simulink model "AvonGasTurbineController"  (R2024b)
settings: Solver=ode45  StartTime=0.0  StopTime=3000  FixedStep=1  RelTol=1e-3  EnableMultiTasking=on
InitFcn:
  | warning off
libraries: slpidlib x3, simulink x2
(part 1 of 2)
settings Model: Creator=Me  LastModifiedBy=argha
settings SolverCC: AlgebraicLoopSolver=TrustRegion
settings DataIOCC: LimitDataPoints=on  SaveFormat=Array  SignalLoggingSaveFormat=ModelDataLogs  ReturnWorkspaceOutputs=off
settings OptimizationCC: ExpressionDepthLimit=2147483647  LifeSpan=inf
settings DebuggingCC: UnderspecifiedInitializationDetection=Classic  MergeDetectMultiDrivingBlocksExec=none  SolverPrmCheckMsg=warning  FcnCallInpInsideContextMsg=warning  UnconnectedInputMsg=warning  UnconnectedOutputMsg=warning  UnconnectedLineMsg=warning  StateNameClashWarn=warning  SFUnexpectedBacktrackingDiag=warning  SFNoUnconditionalDefaultTransitionDiag=warning  SFExecutionAtInitializationDiag=none  ArithmeticOperatorsInVariantConditions=warning
settings HardwareCC: ProdBitPerPointer=32  ProdBitPerSizeT=32  ProdBitPerPtrDiffT=32  ProdLargestAtomicFloat=None  ProdIntDivRoundTo=Undefined  ProdEndianess=Unspecified  ProdWordSize=32  ProdHWDeviceType=32-bit Generic
settings ModelReferenceCC: EnableRefExpFcnMdlSchedulingChecks=on  PropagateSignalLabelsOutOfModel=off
settings SFSimCC: SimUseLocalCustomCode=off  CustomCodeUndefinedFunction=UseInterfaceOnly
settings RTWCC: RTWUseLocalCustomCode=off  GPUComputeCapability=3.5
settings CodeAppCC: StateflowObjectComments=on
settings GRTTargetCC: TargetLangStandard=C89/C90 (ANSI)  CombineOutputUpdateFcns=off  GRTInterface=on
settings ConfigComp: CovMetricSettings=dw  CovSaveCumulativeToWorkspaceVar=on  CovSaveSingleToWorkspaceVar=on  CovExternalEMLEnable=off  CovSFcnEnable=off
settings SimscapeCC: SimscapeNormalizeSystem=off
settings ConfigurationSet: Description=SimMechanics 2G

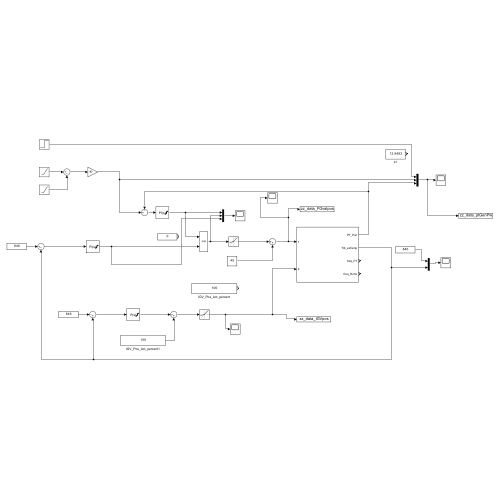
[thumbnail: Simulink's stored preview of the top-level diagram]
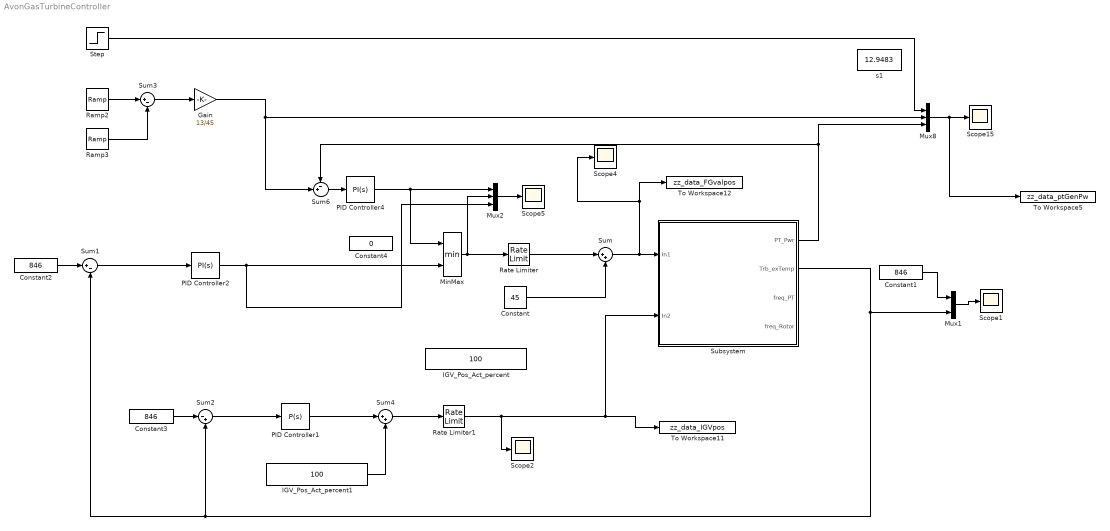
== system AvonGasTurbineController ==
  Constant : Constant  Value=45
  Constant1 : Constant  Value=846
  Constant2 : Constant  Value=846
  Constant3 : Constant  Value=846
  Constant4 : Constant  Value=0
  Gain : Gain  Gain=13/45
  IGV_Pos_Act_percent : Constant  Value=100
  IGV_Pos_Act_percent1 : Constant  Value=100
  MinMax : MinMax  Inputs=2
  Mux1 : Mux  Inputs=2
  Mux2 : Mux  Inputs=3
  Mux8 : Mux  Inputs=3
  PID Controller1 : slpidlib/PID Controller  Controller=P  Form=Ideal  TimeDomain=Continuous-time  UseExternalTs=off  SampleTime=-1  IntegratorMethod=Forward Euler  FilterMethod=Forward Euler  ControllerParametersSource=internal  P=0.1  I=0.180070827922895  UseKiTs=off  D=0  UseExternalDerivativeSource=off  N=100  UseFilter=on  TunerSelectOption=Transfer Function Based (PID Tuner App)  InitialConditionSource=internal  InitialConditionForIntegrator=0  InitialConditionForFilter=0  DifferentiatorICPrevScaledInput=0  ExternalReset=none  TrackingMode=off  Kt=1  LimitOutput=on  SatLimitsSource=internal  UpperSaturationLimit=15  LowerSaturationLimit=-100  LinearizeAsGain=on  AntiWindupMode=back-calculation  Kb=0.2  LimitIntegrator=off  UpperIntegratorSaturationLimit=inf  LowerIntegratorSaturationLimit=-inf  POutMin=[]  POutMax=[]  IOutMin=[]  IOutMax=[]  DOutMin=[]  DOutMax=[]  NOutMin=[]  NOutMax=[]  SumOutMin=[]  SumOutMax=[]  SaturationOutMin=[]  SaturationOutMax=[]  PParamMin=[]  PParamMax=[]  IParamMin=[]  IParamMax=[]  DParamMin=[]  DParamMax=[]  NParamMin=[]  NParamMax=[]  KbParamMin=[]  KbParamMax=[]  KtParamMin=[]  KtParamMax=[]  KbOutMin=[]  KbOutMax=[]  KtOutMin=[]  KtOutMax=[]  IntegratorOutMin=[]  IntegratorOutMax=[]  FilterOutMin=[]  FilterOutMax=[]  SumI1OutMin=[]  SumI1OutMax=[]  SumI2OutMin=[]  SumI2OutMax=[]  SumI3OutMin=[]  SumI3OutMax=[]  SumI4OutMin=[]  SumI4OutMax=[]  SumDOutMin=[]  SumDOutMax=[]  DifferentiatorOutMin=[]  DifferentiatorOutMax=[]  FilterDiffOutCoefMin=[]  FilterDiffOutCoefMax=[]  ReciprocalOutMin=[]  ReciprocalOutMax=[]  SumDenOutMin=[]  SumDenOutMax=[]  SumNumOutMin=[]  SumNumOutMax=[]  DivideOutMin=[]  DivideOutMax=[]  UdiffTsProdOutMin=[]  UdiffTsProdOutMax=[]  NTsProdOutMin=[]  NTsProdOutMax=[]  UintegralTsProdOutMin=[]  UintegralTsProdOutMax=[]  UngainTsProdOutMin=[]  UngainTsProdOutMax=[]  ClampingZeroOutDataTypeStr=Inherit: Inherit via back propagation  ClampingZeroOutMin=[]  ClampingZeroOutMax=[]  FilterDenConstantOutDataTypeStr=Inherit: Inherit via back propagation  FilterDenConstantOutMin=[]  FilterDenConstantOutMax=[]  PCopyOutDataTypeStr=Inherit: Inherit via back propagation  PCopyOutMin=[]  PCopyOutMax=[]  NCopyOutDataTypeStr=Inherit: Inherit via back propagation  NCopyOutMin=[]  NCopyOutMax=[]  IntegratorContinuousStateAttributes=''  IntegratorStateMustResolveToSignalObject=off  IntegratorRTWStateStorageClass=Auto  FilterContinuousStateAttributes=''  FilterStateMustResolveToSignalObject=off  FilterRTWStateStorageClass=Auto  ParallelPVariant=InternalParameters  IdealPVariant=Disabled  IVariant=Disabled  DVariant=Disabled  IntegratorVariant=Disabled  SatVariant=Enabled  AWVariant=Disabled  PCopyVariant=Disabled  TRVariant=Disabled  FdbkBlocksVariant=Forward  IdealPFdbkVariant=Disabled  SatFdbkVariant=Disabled  DerivativeFilterVariant=Disabled  NVariant=Disabled  NCopyVariant=Disabled_SignalSpec  FilterICVariant=Disabled  IntegratorICVariant=Disabled  ExternalResetVariant=Disabled  TRSumVariant=Passthrough  SumFdbkVariant=Disabled  SumVariant=Passthrough_P  TsampFilterVariant=InternalTs  TsampNgainVariant=Passthrough  TsampIntegralVariant=Disabled_SignalSpec  ExternalSaturationOutDataTypeStr=Inherit: Same as second input  DerivativeSourceVariant=Disabled  PreIntVariant=InternalPreInt
  PID Controller2 : slpidlib/PID Controller  Controller=PI  Form=Ideal  TimeDomain=Continuous-time  UseExternalTs=off  SampleTime=-1  IntegratorMethod=Forward Euler  FilterMethod=Forward Euler  ControllerParametersSource=internal  P=0.02  I=0.1  UseKiTs=off  D=0  UseExternalDerivativeSource=off  N=100  UseFilter=on  TunerSelectOption=Transfer Function Based (PID Tuner App)  InitialConditionSource=internal  InitialConditionForIntegrator=20  InitialConditionForFilter=0  DifferentiatorICPrevScaledInput=0  ExternalReset=none  TrackingMode=off  Kt=1  LimitOutput=on  SatLimitsSource=internal  UpperSaturationLimit=45  LowerSaturationLimit=-45  LinearizeAsGain=on  AntiWindupMode=back-calculation  Kb=0.2  LimitIntegrator=off  UpperIntegratorSaturationLimit=inf  LowerIntegratorSaturationLimit=-inf  POutMin=[]  POutMax=[]  IOutMin=[]  IOutMax=[]  DOutMin=[]  DOutMax=[]  NOutMin=[]  NOutMax=[]  SumOutMin=[]  SumOutMax=[]  SaturationOutMin=[]  SaturationOutMax=[]  PParamMin=[]  PParamMax=[]  IParamMin=[]  IParamMax=[]  DParamMin=[]  DParamMax=[]  NParamMin=[]  NParamMax=[]  KbParamMin=[]  KbParamMax=[]  KtParamMin=[]  KtParamMax=[]  KbOutMin=[]  KbOutMax=[]  KtOutMin=[]  KtOutMax=[]  IntegratorOutMin=[]  IntegratorOutMax=[]  FilterOutMin=[]  FilterOutMax=[]  SumI1OutMin=[]  SumI1OutMax=[]  SumI2OutMin=[]  SumI2OutMax=[]  SumI3OutMin=[]  SumI3OutMax=[]  SumI4OutMin=[]  SumI4OutMax=[]  SumDOutMin=[]  SumDOutMax=[]  DifferentiatorOutMin=[]  DifferentiatorOutMax=[]  FilterDiffOutCoefMin=[]  FilterDiffOutCoefMax=[]  ReciprocalOutMin=[]  ReciprocalOutMax=[]  SumDenOutMin=[]  SumDenOutMax=[]  SumNumOutMin=[]  SumNumOutMax=[]  DivideOutMin=[]  DivideOutMax=[]  UdiffTsProdOutMin=[]  UdiffTsProdOutMax=[]  NTsProdOutMin=[]  NTsProdOutMax=[]  UintegralTsProdOutMin=[]  UintegralTsProdOutMax=[]  UngainTsProdOutMin=[]  UngainTsProdOutMax=[]  ClampingZeroOutDataTypeStr=Inherit: Inherit via back propagation  ClampingZeroOutMin=[]  ClampingZeroOutMax=[]  FilterDenConstantOutDataTypeStr=Inherit: Inherit via back propagation  FilterDenConstantOutMin=[]  FilterDenConstantOutMax=[]  PCopyOutDataTypeStr=Inherit: Inherit via back propagation  PCopyOutMin=[]  PCopyOutMax=[]  NCopyOutDataTypeStr=Inherit: Inherit via back propagation  NCopyOutMin=[]  NCopyOutMax=[]  IntegratorContinuousStateAttributes=''  IntegratorStateMustResolveToSignalObject=off  IntegratorRTWStateStorageClass=Auto  FilterContinuousStateAttributes=''  FilterStateMustResolveToSignalObject=off  FilterRTWStateStorageClass=Auto  ParallelPVariant=Passthrough  IdealPVariant=InternalParameters  IVariant=InternalParameters  DVariant=Disabled  IntegratorVariant=Continuous  SatVariant=Enabled  AWVariant=BackCalculation  PCopyVariant=Disabled  TRVariant=Disabled  FdbkBlocksVariant=Forward  IdealPFdbkVariant=Disabled  SatFdbkVariant=Disabled  DerivativeFilterVariant=Disabled  NVariant=Disabled  NCopyVariant=Disabled_SignalSpec  FilterICVariant=Disabled  IntegratorICVariant=InternalICs  ExternalResetVariant=Disabled  TRSumVariant=Passthrough  SumFdbkVariant=Disabled  SumVariant=Sum_PI  TsampFilterVariant=InternalTs  TsampNgainVariant=Passthrough  TsampIntegralVariant=Disabled_SignalSpec  ExternalSaturationOutDataTypeStr=Inherit: Same as second input  DerivativeSourceVariant=Disabled  PreIntVariant=InternalPreInt
  PID Controller4 : slpidlib/PID Controller  Controller=PI  Form=Ideal  TimeDomain=Continuous-time  UseExternalTs=off  SampleTime=-1  IntegratorMethod=Forward Euler  FilterMethod=Forward Euler  ControllerParametersSource=internal  P=0.17  I=0.2  UseKiTs=off  D=0  UseExternalDerivativeSource=off  N=100  UseFilter=on  TunerSelectOption=Transfer Function Based (PID Tuner App)  InitialConditionSource=internal  InitialConditionForIntegrator=0  InitialConditionForFilter=0  DifferentiatorICPrevScaledInput=0  ExternalReset=none  TrackingMode=off  Kt=1  LimitOutput=on  SatLimitsSource=internal  UpperSaturationLimit=60  LowerSaturationLimit=-30  LinearizeAsGain=on  AntiWindupMode=back-calculation  Kb=0.2  LimitIntegrator=off  UpperIntegratorSaturationLimit=inf  LowerIntegratorSaturationLimit=-inf  POutMin=[]  POutMax=[]  IOutMin=[]  IOutMax=[]  DOutMin=[]  DOutMax=[]  NOutMin=[]  NOutMax=[]  SumOutMin=[]  SumOutMax=[]  SaturationOutMin=[]  SaturationOutMax=[]  PParamMin=[]  PParamMax=[]  IParamMin=[]  IParamMax=[]  DParamMin=[]  DParamMax=[]  NParamMin=[]  NParamMax=[]  KbParamMin=[]  KbParamMax=[]  KtParamMin=[]  KtParamMax=[]  KbOutMin=[]  KbOutMax=[]  KtOutMin=[]  KtOutMax=[]  IntegratorOutMin=[]  IntegratorOutMax=[]  FilterOutMin=[]  FilterOutMax=[]  SumI1OutMin=[]  SumI1OutMax=[]  SumI2OutMin=[]  SumI2OutMax=[]  SumI3OutMin=[]  SumI3OutMax=[]  SumI4OutMin=[]  SumI4OutMax=[]  SumDOutMin=[]  SumDOutMax=[]  DifferentiatorOutMin=[]  DifferentiatorOutMax=[]  FilterDiffOutCoefMin=[]  FilterDiffOutCoefMax=[]  ReciprocalOutMin=[]  ReciprocalOutMax=[]  SumDenOutMin=[]  SumDenOutMax=[]  SumNumOutMin=[]  SumNumOutMax=[]  DivideOutMin=[]  DivideOutMax=[]  UdiffTsProdOutMin=[]  UdiffTsProdOutMax=[]  NTsProdOutMin=[]  NTsProdOutMax=[]  UintegralTsProdOutMin=[]  UintegralTsProdOutMax=[]  UngainTsProdOutMin=[]  UngainTsProdOutMax=[]  ClampingZeroOutDataTypeStr=Inherit: Inherit via back propagation  ClampingZeroOutMin=[]  ClampingZeroOutMax=[]  FilterDenConstantOutDataTypeStr=Inherit: Inherit via back propagation  FilterDenConstantOutMin=[]  FilterDenConstantOutMax=[]  PCopyOutDataTypeStr=Inherit: Inherit via back propagation  PCopyOutMin=[]  PCopyOutMax=[]  NCopyOutDataTypeStr=Inherit: Inherit via back propagation  NCopyOutMin=[]  NCopyOutMax=[]  IntegratorContinuousStateAttributes=''  IntegratorStateMustResolveToSignalObject=off  IntegratorRTWStateStorageClass=Auto  FilterContinuousStateAttributes=''  FilterStateMustResolveToSignalObject=off  FilterRTWStateStorageClass=Auto  ParallelPVariant=Passthrough  IdealPVariant=InternalParameters  IVariant=InternalParameters  DVariant=Disabled  IntegratorVariant=Continuous  SatVariant=Enabled  AWVariant=BackCalculation  PCopyVariant=Disabled  TRVariant=Disabled  FdbkBlocksVariant=Forward  IdealPFdbkVariant=Disabled  SatFdbkVariant=Disabled  DerivativeFilterVariant=Disabled  NVariant=Disabled  NCopyVariant=Disabled_SignalSpec  FilterICVariant=Disabled  IntegratorICVariant=InternalICs  ExternalResetVariant=Disabled  TRSumVariant=Passthrough  SumFdbkVariant=Disabled  SumVariant=Sum_PI  TsampFilterVariant=InternalTs  TsampNgainVariant=Passthrough  TsampIntegralVariant=Disabled_SignalSpec  ExternalSaturationOutDataTypeStr=Inherit: Same as second input  DerivativeSourceVariant=Disabled  PreIntVariant=InternalPreInt
  Ramp2 : simulink/Sources/Ramp  slope=0.05  start=1500  InitialOutput=30
  Ramp3 : simulink/Sources/Ramp  slope=0.05  start=1800  InitialOutput=0
  Rate Limiter : RateLimiter  RisingSlewLimit=0.1  FallingSlewLimit=-0.1  SampleTimeMode=inherited  InitialCondition=45
  Rate Limiter1 : RateLimiter  RisingSlewLimit=0.1  FallingSlewLimit=-0.1  SampleTimeMode=inherited  InitialCondition=45
  Scope{1..2,4..5,15} (5 alike) : Scope
  Step : Step  Time=1500  Before=8.66  After=13  SampleTime=0
  Subsystem : Subsystem
  Sum : Sum  Inputs=|++
  Sum1 : Sum  Inputs=|+-
  Sum2 : Sum  Inputs=|-+
  Sum3 : Sum  Inputs=|+-
  Sum4 : Sum  Inputs=|++
  Sum6 : Sum  Inputs=-+|
  To Workspace11 : ToWorkspace  VariableName=zz_data_IGVpos  SampleTime=1
  To Workspace12 : ToWorkspace  VariableName=zz_data_FGvalpos  SampleTime=1
  To Workspace5 : ToWorkspace  VariableName=zz_data_ptGenPw  SampleTime=1
  s1 : Constant  Value=12.9483
  wires:
  Ramp3/1 -> Sum3/2
  Ramp2/1 -> Sum3/1
  Subsystem/2(Trb_exTemp) -> Mux1/2, Sum2/2, Sum1/2
  Sum3/1 -> Gain/1
  Sum6/1 -> PID Controller4/1
  Constant2/1 -> Sum1/1
  PID Controller2/1 -> Mux2/3, MinMax/2
  PID Controller4/1 -> Mux2/1, MinMax/1
  Gain/1 -> Mux8/2, Sum6/2
  Constant/1 -> Sum/2
  Sum/1 -> Scope4/1, To Workspace12/1, Subsystem/1(In1)
  MinMax/1 -> Mux2/2, Rate Limiter/1
  Mux1/1 -> Scope1/1
  Constant1/1 -> Mux1/1
  Sum2/1 -> PID Controller1/1
  Constant3/1 -> Sum2/1
  PID Controller1/1 -> Sum4/1
  IGV_Pos_Act_percent1/1 -> Sum4/2
  Sum4/1 -> Rate Limiter1/1
  Rate Limiter1/1 -> Subsystem/2(In2), To Workspace11/1, Scope2/1
  Mux8/1 -> To Workspace5/1, Scope15/1
  Subsystem/1(PT_Pwr) -> Mux8/3, Sum6/1
  Step/1 -> Mux8/1
  Sum1/1 -> PID Controller2/1
  Rate Limiter/1 -> Sum/1
  Mux2/1 -> Scope5/1

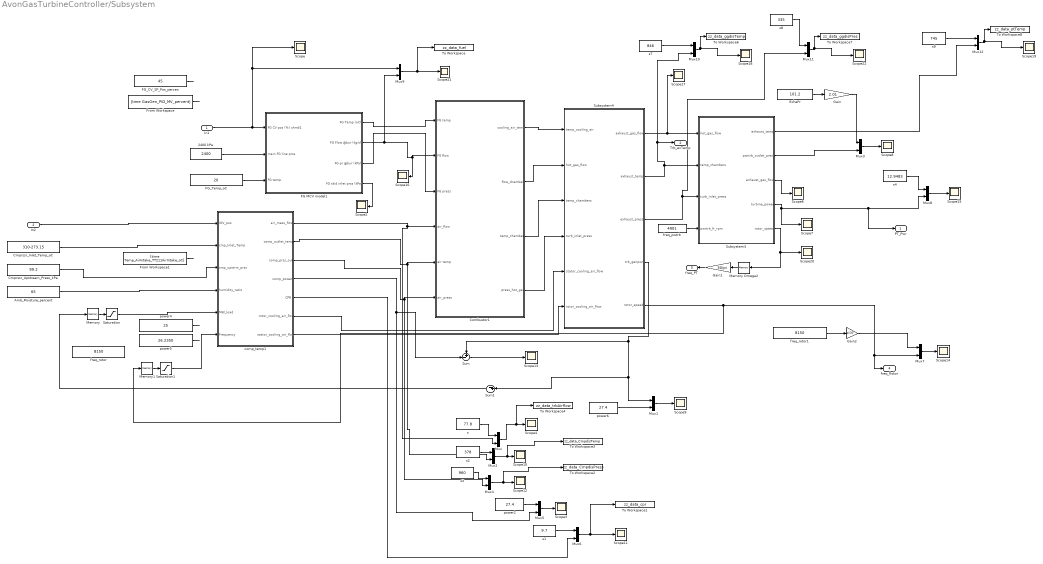
== system AvonGasTurbineController/Subsystem ==
  In1 : Inport
  In2 : Inport  Port=2
  2400 kPa : Constant  Value=2400
  Amb_Moisture_percent : Constant  Value=65
  Cmprssr_Inlet_Temp_oC : Constant  Value=310-273.15
  Cmprssr_Upstream_Press_kPa : Constant  Value=99.2
  Combustor1 : Subsystem
  ExhaPr : Constant  Value=101.2
  FG MCV model1 : Subsystem
  FG_CV_SP_Pos_percen : Constant  Value=45
  FG_Temp_oC : Constant  Value=20
  From Workspace : FromWorkspace  VariableName=[time GasGen_PID_MV_percent]
  From Workspace1 : FromWorkspace  VariableName="[time  Temp_AirIntake_TT211AirIntake_oC]"
  Gain : Gain  Gain=2.01
  Gain1 : Gain  Gain=30/pi
  Gain2 : Gain  Gain=pi/30
  Memory : Memory  InitialCondition=28.945
  Memory Omega2 : Memory  InitialCondition=pi/30*4901
  Memory1 : Memory  InitialCondition=8150
  Mux{,1..12} (13 alike) : Mux  Inputs=2
  Saturation : Saturate  UpperLimit=40  LowerLimit=1
  Saturation1 : Saturate  UpperLimit=8300  LowerLimit=7000
  Scope{,2..4,6..22} (21 alike) : Scope
  Subsystem3 : Subsystem
  Subsystem4 : Subsystem
  Sum : Sum  Inputs=+-|
  Sum1 : Sum  Inputs=-+|
  To Workspace : ToWorkspace  VariableName=zz_data_fuel  SaveFormat=Timeseries  SampleTime=1
  To Workspace1 : ToWorkspace  VariableName=zz_data_cpr  SampleTime=1
  To Workspace2 : ToWorkspace  VariableName=zz_data_CmpdisPress  SampleTime=1
  To Workspace3 : ToWorkspace  VariableName=zz_data_CmpdisTemp  SaveFormat=Timeseries  SampleTime=1
  To Workspace4 : ToWorkspace  VariableName=zz_data_trbAirflow  SampleTime=1
  To Workspace6 : ToWorkspace  VariableName=zz_data_ggdisTemp  SampleTime=1
  To Workspace7 : ToWorkspace  VariableName=zz_data_ggdisPres  SampleTime=1
  To Workspace8 : ToWorkspace  VariableName=zz_data_ptTemp  SampleTime=1
  comp_temp1 : Subsystem
  freq_pwtrb : Constant  Value=4901
  freq_rotor : Constant  Value=8150
  freq_rotor1 : Constant  Value=8150
  power2 : Constant  Value=27.4
  power4 : Constant  Value=25
  power5 : Constant  Value=26.2350
  power6 : Constant  Value=27.4
  s : Constant  Value=77.8
  s1 : Constant  Value=9.7
  s2 : Constant  Value=378
  s3 : Constant  Value=960
  s4 : Constant  Value=12.9483
  s7 : Constant  Value=846
  s8 : Constant  Value=335
  s9 : Constant  Value=745
  PT_Pwr : Outport
  Trb_exTemp : Outport  Port=2
  freq_PT : Outport  Port=3
  freq_Rotor : Outport  Port=4
  wires:
  FG_CV_SP_Pos_percen/1 -> ?
  From Workspace/1 -> ?
  Gain1/1 -> freq_PT/1
  From Workspace1/1 -> ?
  power5/1 -> ?
  power4/1 -> ?
  Subsystem4/2(exhaust_temp) -> Subsystem3/2(temp_chambers), Trb_exTemp/1, Mux10/2
  Cmprssr_Upstream_Press_kPa/1 -> comp_temp1/3(cmp_upstrm_prss)
  Amb_Moisture_percent/1 -> comp_temp1/4(humidity_ratio)
  Saturation1/1 -> comp_temp1/6(Frequency)
  In2/1 -> comp_temp1/1(IGV_pos)
  Subsystem3/3(exhaust_gas_flow) -> Scope6/1
  Memory/1 -> Saturation/1
  FG_Temp_oC/1 -> FG MCV model1/3(FG temp.)
  comp_temp1/3(comp_prss_out) -> Mux4/2, Combustor1/6(air_press)
  FG MCV model1/2(FG Flow @bur (kg/s)) -> Mux9/2, Scope16/1, Combustor1/2(FG flow)
  Combustor1/2(flow_chamber) -> Subsystem4/2(hot_gas_flow)
  comp_temp1/4(comp_power) -> Mux5/2, Sum/2
  Mux1/1 -> Scope9/1
  Mux6/1 -> To Workspace1/1, Scope11/1
  comp_temp1/5(CPR) -> Mux6/2
  Mux4/1 -> To Workspace2/1, Scope12/1
  FG MCV model1/1(FG Temp (oC)) -> Combustor1/1(FG temp)
  Mux2/1 -> To Workspace3/1, Scope10/1
  2400 kPa/1 -> FG MCV model1/2(main FG line prss)
  ExhaPr/1 -> Gain/1
  Combustor1/1(cooling_air_temp) -> Subsystem4/1(temp_cooling_air)
  FG MCV model1/3(FG pr @bur (kPa)) -> Combustor1/3(FG press)
  Subsystem4/3(exhaust_press) -> Mux11/2, Subsystem3/3(turb_inlet_press)
  Combustor1/3(temp_chamber) -> Subsystem4/3(temp_chambers)
  FG MCV model1/4(FG skid inlet prss (kPa)) -> Scope2/1
  Subsystem4/1(exhaust_gas_flow) -> Scope17/1, Subsystem3/1(hot_gas_flow)
  Subsystem3/2(pwrtrb_outlet_press) -> Mux3/2
  power6/1 -> Mux1/2
  Gain/1 -> Mux3/1
  Mux3/1 -> Scope8/1
  comp_temp1/1(air_mass_flow) -> Mux/2, Combustor1/4(air_flow)
  Subsystem3/1(exhaust_temp) -> Mux12/2
  comp_temp1/2(comp_outlet_temp) -> Mux2/2, Combustor1/5(air temp)
  Combustor1/4(press_hot_gas) -> Subsystem4/4(turb_inlet_press)
  Mux8/1 -> Scope15/1
  Mux7/1 -> Scope14/1
  In1/1 -> Mux9/1, Scope/1, FG MCV model1/1(FG CV pos (%) chmb1)
  Subsystem3/4(turbine_power) -> PT_Pwr/1, Mux8/2, Scope7/1
  comp_temp1/7(stator_cooling_air_flow) -> Subsystem4/6(rotor_cooling_air_flow)
  Cmprssr_Inlet_Temp_oC/1 -> comp_temp1/2(cmp_Inlet_Temp)
  Mux11/1 -> To Workspace7/1, Scope22/1
  s2/1 -> Mux2/1
  Sum1/1 -> Memory/1
  Mux9/1 -> To Workspace/1, Scope21/1
  Mux/1 -> To Workspace4/1, Scope4/1
  s/1 -> Mux/1
  s7/1 -> Mux10/1
  s1/1 -> Mux6/1
  Mux10/1 -> Scope18/1, To Workspace6/1
  Mux5/1 -> Scope3/1
  Sum/1 -> Scope13/1
  Subsystem4/5(rotor_speed) -> Memory1/1, freq_Rotor/1, Mux7/2
  comp_temp1/6(rotor_cooling_air_flow) -> Subsystem4/5(stator_cooling_air_flow)
  s3/1 -> Mux4/1
  freq_pwtrb/1 -> Subsystem3/4(pwrtrb_fr_rpm)
  power2/1 -> Mux5/1
  Subsystem3/5(rotor_speed) -> Scope20/1, Memory Omega2/1
  Gain2/1 -> Mux7/1
  Saturation/1 -> comp_temp1/5(MW_load)
  Memory Omega2/1 -> Gain1/1
  freq_rotor1/1 -> Gain2/1
  Subsystem4/4(trb_genpwr) -> Sum/1, Sum1/2, Mux1/1
  s4/1 -> Mux8/1
  s9/1 -> Mux12/1
  s8/1 -> Mux11/1
  Mux12/1 -> To Workspace8/1, Scope19/1
  Memory1/1 -> Saturation1/1

== system AvonGasTurbineController/Subsystem/Combustor1 ==
  FG temp : Inport
  FG flow : Inport  Port=2
  FG press : Inport  Port=3
  air_flow : Inport  Port=4
  air temp : Inport  Port=5
  air_press : Inport  Port=6
  Scope1 : Scope
  Scope2 : Scope
  Scope3 : Scope
  combustion chamber 1 : Subsystem
  cooling_air_temp : Outport
  flow_chamber : Outport  Port=2
  temp_chamber : Outport  Port=3
  press_hot_gas : Outport  Port=4
  wires:
  FG flow/1 -> combustion chamber 1/1(Fg flow)
  FG press/1 -> combustion chamber 1/2(FG press)
  FG temp/1 -> combustion chamber 1/3(FG temp)
  combustion chamber 1/1(temp chamber 1) -> Scope1/1, temp_chamber/1
  air_press/1 -> combustion chamber 1/6(air_press)
  air temp/1 -> Scope2/1, cooling_air_temp/1, combustion chamber 1/5(air_temp)
  combustion chamber 1/2(flow) -> Scope3/1, flow_chamber/1
  air_flow/1 -> combustion chamber 1/4(air flow)
  combustion chamber 1/3(Gas_press) -> press_hot_gas/1

== system AvonGasTurbineController/Subsystem/FG MCV model1 ==
  FG CV pos (%) chmb1 : Inport
  main FG line prss : Inport  Port=2
  FG temp. : Inport  Port=3
  " Memory " : Memory  InitialCondition=1.9
  CV model chamber 2 : Subsystem
  Subsystem1 : Subsystem
  FG Temp (oC) : Outport
  FG Flow @bur (kg/s) : Outport  Port=2
  FG pr @bur (kPa) : Outport  Port=3
  FG skid inlet prss (kPa) : Outport  Port=4
  tag scope: FG_flow=global
  wires:
  Subsystem1/2(skid temp) -> CV model chamber 2/3(FG temp.)
  " Memory "/1 -> Subsystem1/3(FG flow)
  main FG line prss/1 -> Subsystem1/1(gas prss)
  Subsystem1/1(" FG skid inlet prss") -> CV model chamber 2/2(Skid inlet prss), FG skid inlet prss (kPa)/1
  FG temp./1 -> Subsystem1/2(FG temp.), FG Temp (oC)/1
  CV model chamber 2/1(FG pr @bur) -> FG pr @bur (kPa)/1
  FG CV pos (%) chmb1/1 -> CV model chamber 2/1(FG valve pos.)
  CV model chamber 2/2(FG flow) -> FG Flow @bur (kg/s)/1, [FG_flow], " Memory "/1

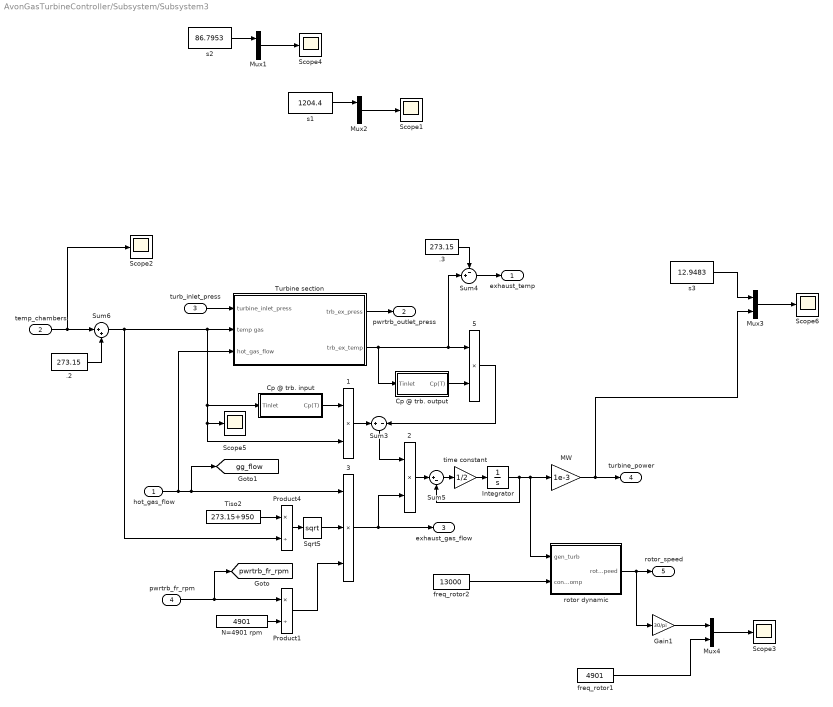
== system AvonGasTurbineController/Subsystem/Subsystem3 ==
  hot_gas_flow : Inport
  temp_chambers : Inport  Port=2
  turb_inlet_press : Inport  Port=3
  pwrtrb_fr_rpm : Inport  Port=4
  "    .2" : Constant  Value=273.15
  "    .3" : Constant  Value=273.15
  " 1" : Product  RndMeth=Zero
  " 2" : Product  RndMeth=Zero
  " 3" : Product  Inputs=3  RndMeth=Zero
  " 5" : Product  RndMeth=Zero
  Cp @ trb. input : Subsystem
  Cp @ trb. output : Subsystem
  Gain1 : Gain  Gain=30/pi
  Integrator : Integrator  InitialCondition=13000  LimitOutput=on  UpperSaturationLimit=20000  LowerSaturationLimit=1
  MW : Gain  Gain=1e-3
  Mux1 : Mux  Inputs=2
  Mux2 : Mux  Inputs=3
  Mux3 : Mux  Inputs=2
  Mux4 : Mux  Inputs=2
  N=4901 rpm : Constant  Value=4901
  Product1 : Product  Inputs=*/  RndMeth=Zero
  Product4 : Product  Inputs=*/  RndMeth=Zero
  Scope{1..6} (6 alike) : Scope
  Sqrt5 : Sqrt
  Sum3 : Sum  Inputs=+-
  Sum4 : Sum  Inputs=-+|
  Sum5 : Sum  Inputs=|+-
  Sum6 : Sum  Inputs=|++
  Tiso2 : Constant  Value=273.15+950
  Turbine section : Subsystem
  freq_rotor1 : Constant  Value=4901
  freq_rotor2 : Constant  Value=13000
  rotor dynamic : Subsystem
  s1 : Constant  Value=1204.4
  s2 : Constant  Value=86.7953
  s3 : Constant  Value=12.9483
  time constant : Gain  Gain=1/2
  exhaust_temp : Outport
  pwrtrb_outlet_press : Outport  Port=2
  exhaust_gas_flow : Outport  Port=3
  turbine_power : Outport  Port=4
  rotor_speed : Outport  Port=5
  tag scope: gg_flow=global, pwrtrb_fr_rpm=global
  wires:
  Turbine section/2(trb_ex_temp) -> " 5"/1, Sum4/2, Cp @ trb. output/1(Tinlet)
  s3/1 -> Mux3/1
  Mux3/1 -> Scope6/1
  turb_inlet_press/1 -> Turbine section/1(turbine_inlet_press)
  "    .3"/1 -> Sum4/1
  Sum4/1 -> exhaust_temp/1
  temp_chambers/1 -> Scope2/1, Sum6/1
  "    .2"/1 -> Sum6/2
  s1/1 -> Mux2/1
  Mux2/1 -> Scope1/1
  s2/1 -> Mux1/1
  Mux1/1 -> Scope4/1
  " 2"/1 -> Sum5/1
  " 5"/1 -> Sum3/2
  Cp @ trb. output/1(Cp(T)) -> " 5"/2
  Cp @ trb. input/1(Cp(T)) -> " 1"/1
  time constant/1 -> Integrator/1
  Sum5/1 -> time constant/1
  " 1"/1 -> Sum3/1
  Sum3/1 -> " 2"/1
  Tiso2/1 -> Product4/1
  Sum6/1 -> Product4/2, Cp @ trb. input/1(Tinlet), " 1"/2, Scope5/1, Turbine section/2(temp gas)
  Product4/1 -> Sqrt5/1
  N=4901 rpm/1 -> Product1/2
  pwrtrb_fr_rpm/1 -> [pwrtrb_fr_rpm], Product1/1
  Product1/1 -> " 3"/3
  Sqrt5/1 -> " 3"/2
  hot_gas_flow/1 -> Turbine section/3(hot_gas_flow), [gg_flow], " 3"/1
  " 3"/1 -> exhaust_gas_flow/1, " 2"/2
  Turbine section/1(trb_ex_press) -> pwrtrb_outlet_press/1
  rotor dynamic/1(rotor_speed) -> Gain1/1, rotor_speed/1
  Integrator/1 -> Sum5/2, MW/1, rotor dynamic/1(gen_turb)
  MW/1 -> turbine_power/1, Mux3/2
  Mux4/1 -> Scope3/1
  freq_rotor1/1 -> Mux4/2
  Gain1/1 -> Mux4/1
  freq_rotor2/1 -> rotor dynamic/2(consm_comp)

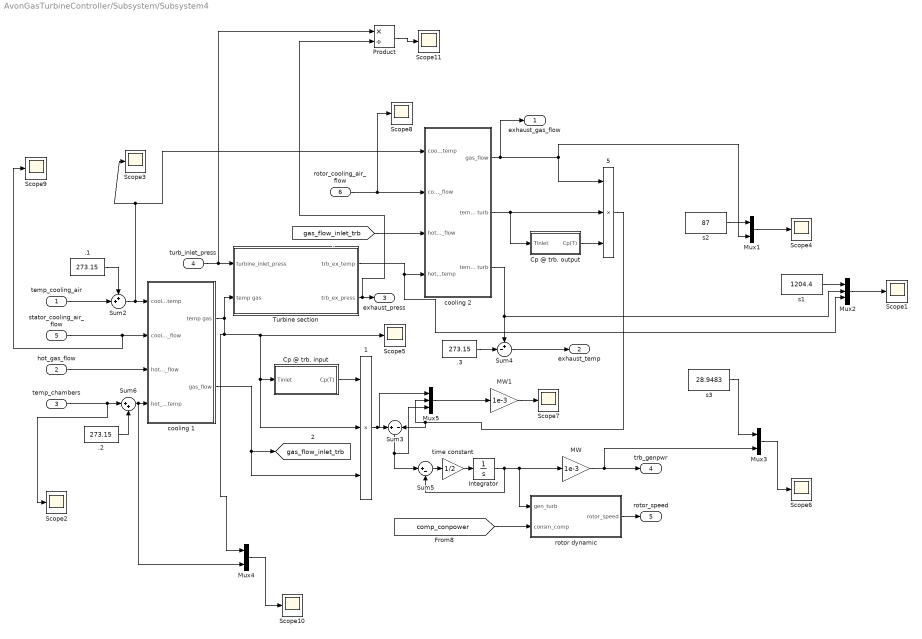
== system AvonGasTurbineController/Subsystem/Subsystem4 ==
  temp_cooling_air : Inport
  hot_gas_flow : Inport  Port=2
  temp_chambers : Inport  Port=3
  turb_inlet_press : Inport  Port=4
  stator_cooling_air_flow : Inport  Port=5
  rotor_cooling_air_flow : Inport  Port=6
  "    .1" : Constant  Value=273.15
  "    .2" : Constant  Value=273.15
  "    .3" : Constant  Value=273.15
  " 1" : Product  Inputs=3  RndMeth=Zero
  " 5" : Product  Inputs=3  RndMeth=Zero
  Cp @ trb. input : Subsystem
  Cp @ trb. output : Subsystem
  Integrator : Integrator  InitialCondition=13500  LimitOutput=on  UpperSaturationLimit=34000  LowerSaturationLimit=10
  MW : Gain  Gain=1e-3
  MW1 : Gain  Gain=1e-3
  Mux1 : Mux  Inputs=2
  Mux2 : Mux  Inputs=3
  Mux3 : Mux  Inputs=2
  Mux4 : Mux  Inputs=2
  Mux5 : Mux  Inputs=3
  Product : Product  Inputs=*/
  Scope{1..11} (11 alike) : Scope
  Sum2 : Sum  Inputs=++|
  Sum3 : Sum  Inputs=+-
  Sum4 : Sum  Inputs=+-|
  Sum5 : Sum  Inputs=|+-
  Sum6 : Sum  Inputs=|++
  Turbine section : Subsystem
  cooling 1 : Subsystem
  cooling 2 : Subsystem
  "rotor dynamic " : Subsystem
  s1 : Constant  Value=1204.4
  s2 : Constant  Value=87
  s3 : Constant  Value=28.9483
  time constant : Gain  Gain=1/2
  exhaust_gas_flow : Outport
  exhaust_temp : Outport  Port=2
  exhaust_press : Outport  Port=3
  trb_genpwr : Outport  Port=4
  rotor_speed : Outport  Port=5
  tag scope: gas_flow_inlet_trb=global
  wires:
  Sum2/1 -> cooling 1/1(cooling_air_temp), cooling 2/1(cooling_air_temp), Scope3/1
  hot_gas_flow/1 -> cooling 1/3(hot_gas_flow)
  " 1"/1 -> Mux5/1, Sum3/1
  rotor_cooling_air_flow/1 -> Scope8/1, cooling 2/2(cooling_air_flow)
  Sum5/1 -> time constant/1
  time constant/1 -> Integrator/1
  [gas_flow_inlet_trb] -> cooling 2/3(hot_gas_flow)
  Cp @ trb. input/1(Cp(T)) -> " 1"/1
  Turbine section/1(trb_ex_temp) -> Mux2/3, cooling 2/4(hot_gas_temp)
  cooling 2/3(temp exh turb) -> Mux2/2, Sum4/1
  Cp @ trb. output/1(Cp(T)) -> " 5"/3
  " 5"/1 -> Sum3/2, Mux5/2
  cooling 1/2(gas_flow) -> " 1"/3, [gas_flow_inlet_trb]
  Sum3/1 -> Mux5/3, Sum5/1
  Mux1/1 -> Scope4/1
  s2/1 -> Mux1/1
  cooling 2/1(gas_flow) -> " 5"/1, Mux1/2, exhaust_gas_flow/1
  Mux2/1 -> Scope1/1
  s1/1 -> Mux2/1
  "    .1"/1 -> Sum2/1
  temp_cooling_air/1 -> Sum2/2
  "    .2"/1 -> Sum6/2
  temp_chambers/1 -> Scope2/1, Sum6/1
  Sum4/1 -> exhaust_temp/1
  "    .3"/1 -> Sum4/2
  turb_inlet_press/1 -> Product/1, Turbine section/1(turbine_inlet_press)
  Mux3/1 -> Scope6/1
  s3/1 -> Mux3/1
  Integrator/1 -> "rotor dynamic "/1(gen_turb), MW/1, Sum5/2
  cooling 2/2(temp turb) -> Cp @ trb. output/1(Tinlet), " 5"/2
  Turbine section/2(trb_ex_press) -> Product/2, exhaust_press/1
  MW/1 -> Mux3/2, trb_genpwr/1
  [comp_conpower] -> "rotor dynamic "/2(consm_comp)
  "rotor dynamic "/1(rotor_speed) -> rotor_speed/1
  stator_cooling_air_flow/1 -> cooling 1/2(cooling_air_flow), Scope9/1
  Mux4/1 -> Scope10/1
  cooling 1/1(temp gas) -> Turbine section/2(temp gas), Cp @ trb. input/1(Tinlet), " 1"/2, Scope5/1, Mux4/1
  Sum6/1 -> Mux4/2, cooling 1/4(hot_gas_temp)
  Mux5/1 -> MW1/1
  MW1/1 -> Scope7/1
  Product/1 -> Scope11/1

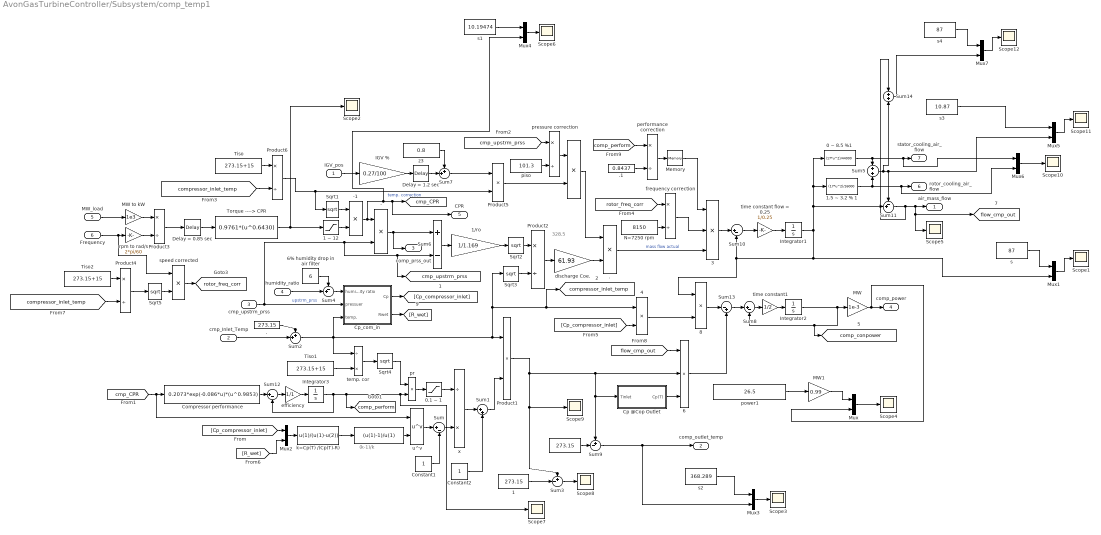
== system AvonGasTurbineController/Subsystem/comp_temp1 ==
  note: (k-1)/k
  note: 328.5
  IGV_pos : Inport
  cmp_Inlet_Temp : Inport  Port=2
  cmp_upstrm_prss : Inport  Port=3
  humidity_ratio : Inport  Port=4
  MW_load : Inport  Port=5
  Frequency : Inport  Port=6
  " " : Fcn  Expr=(u(1)-1)/u(1)
  "    " : Constant  Value=273.15
  "     " : Product  RndMeth=Zero
  "    1" : Constant  Value=273.15
  " 1.5 ~ 3.2 % 1" : Fcn  Expr=(17*u^2)/16000  SampleTime=1
  " 3" : Product  Inputs=3  RndMeth=Zero
  " 4" : Product  RndMeth=Zero
  " 6" : Product  Inputs=3  RndMeth=Zero
  " 8" : Product  RndMeth=Zero
  - : Product  RndMeth=Zero
  -1 : Product  RndMeth=Zero
  . : Constant  Value=273.15
  ". " : Product  RndMeth=Zero
  .1 : Constant  Value=0.8437
  0 ~ 8.5 %1 : Fcn  Expr=(17*u^2)/44000  SampleTime=1
  0.1 ~ 1 : Saturate  UpperLimit=1  LowerLimit=0.1
  1 ~ 12 : Saturate  UpperLimit=20  LowerLimit=1
  1/ro : Gain  Gain=1/1.169
  6% humidity drop in air filter : Constant  Value=6
  "Compressor performance " : Fcn  Expr=0.2073*exp(-0.086*u)*(u^0.9853)
  Constant1 : Constant
  Constant2 : Constant
  Cp @Cop Outlet : Subsystem
  Cp_com_in : Subsystem
  Delay = 0.85 sec : TransportDelay  DelayTime=0.85  InitialOutput=10.706
  Delay = 1.2 sec : TransportDelay  DelayTime=1.2  InitialOutput=0.27
  IGV % : Gain  Gain=0.27/100
  Integrator1 : Integrator  InitialCondition=87  LimitOutput=on  UpperSaturationLimit=140  LowerSaturationLimit=1
  Integrator2 : Integrator  InitialCondition=28000  LimitOutput=on  UpperSaturationLimit=32000  LowerSaturationLimit=10
  Integrator3 : Integrator  InitialCondition=0.6  LimitOutput=on  UpperSaturationLimit=1  LowerSaturationLimit=0
  MW : Gain  Gain=1e-3
  MW to kW : Gain  Gain=1e3
  MW1 : Gain  Gain=0.99
  Memory : Memory  InitialCondition=1.5
  Mux{,1..7} (8 alike) : Mux  Inputs=2
  N=7250 rpm : Constant  Value=8150
  Product1 : Product  RndMeth=Zero
  Product{2..4,6} (4 alike) : Product  Inputs=*/  RndMeth=Zero
  Product5 : Product  RndMeth=Zero
  Scope{1..12} (12 alike) : Scope
  Sqrt{1..5} (5 alike) : Sqrt
  Sum{,8,10,12} (4 alike) : Sum  Inputs=|+-
  Sum1 : Sum  Inputs=|++
  Sum11 : Sum  Inputs=-+|
  Sum13 : Sum  Inputs=|-+
  Sum14 : Sum
  Sum2 : Sum  Inputs=++|
  Sum3 : Sum  Inputs=+-|
  Sum4 : Sum  Inputs=-+|
  Sum5 : Sum
  Sum6 : Sum  Inputs=+-
  Sum7 : Sum  Inputs=++|
  Sum9 : Sum  Inputs=+-|
  Tiso : Constant  Value=273.15+15
  Tiso1 : Constant  Value=273.15+15
  Tiso2 : Constant  Value=273.15+15
  Torque ----> CPR : Fcn  Expr=0.9761*(u^0.6430)
  "discharge Coe. " : Gain  Gain=61.93
  efficiency : Gain  Gain=1/1
  frequency correction : Product  Inputs=*/  RndMeth=Zero
  k=Cp(T) /(Cp(T)-R) : Fcn  Expr=u(1)/(u(1)-u(2))
  performance correction : Product  Inputs=*/  RndMeth=Zero
  piso : Constant  Value=101.3
  power1 : Constant  Value=26.5
  "pr " : Product  RndMeth=Zero
  pressure correction : Product  Inputs=*/  RndMeth=Zero
  rpm to rad/s : Gain  Gain=2*pi/60
  s : Constant  Value=87
  s1 : Constant  Value=10.19474
  s2 : Constant  Value=368.289
  s3 : Constant  Value=10.87
  s4 : Constant  Value=87
  speed corrected : Product  RndMeth=Zero
  temp. cor : Product  Inputs=/*  RndMeth=Zero
  time constant flow = 0.25 : Gain  Gain=1/0.25
  time constant1 : Gain  Gain=1/2
  u^v : Math  Operator=pow  SignedPower=on
  x : Product  Inputs=/*  RndMeth=Zero
  z3 : Constant  Value=0.8
  air_mass_flow : Outport
  comp_outlet_temp : Outport  Port=2
  comp_prss_out : Outport  Port=3
  comp_power : Outport  Port=4
  CPR : Outport  Port=5
  rotor_cooling_air_flow : Outport  Port=6
  stator_cooling_air_flow : Outport  Port=7
  tag scope: cmp_CPR=global, cmp_upstrm_prss=global, comp_conpower=global, comp_perform=global, compressor_inlet_temp=global, flow_cmp_out=global, rotor_freq_corr=global
  wires:
  [cmp_CPR] -> "Compressor performance "/1, u^v/1
  " "/1 -> u^v/2
  u^v/1 -> Sum/1
  Sum/1 -> x/2
  Constant2/1 -> Sum1/2
  Sum1/1 -> Product1/2
  Sum2/1 -> Cp_com_in/3(temp.), Product1/1, Sqrt3/1, [compressor_inlet_temp], " 4"/1, temp. cor/1
  x/1 -> Sum1/1
  Constant1/1 -> Sum/2
  cmp_upstrm_prss/1 -> Cp_com_in/2(pressuer), -/2, Sum6/2, [cmp_upstrm_prss]  "upstrm_prss"
  cmp_Inlet_Temp/1 -> Sum2/2
  "Compressor performance "/1 -> Sum12/1
  0.1 ~ 1/1 -> x/1
  k=Cp(T) /(Cp(T)-R)/1 -> " "/1
  Cp_com_in/1(Cp) -> [Cp_compressor_inlet]
  Sum4/1 -> Cp_com_in/1(humidity ratio)
  humidity_ratio/1 -> Sum4/2
  6% humidity drop in air filter/1 -> Sum4/1
  -/1 -> comp_prss_out/1, Sum6/1
  Frequency/1 -> speed corrected/1, rpm to rad/s/1
  Sum6/1 -> 1/ro/1
  1/ro/1 -> Sqrt2/1
  Sqrt3/1 -> Product2/2
  Product2/1 -> "discharge Coe. "/1
  Sqrt2/1 -> Product2/1
  IGV_pos/1 -> IGV %/1
  piso/1 -> pressure correction/2
  [cmp_upstrm_prss] -> pressure correction/1
  Product5/1 -> "     "/2
  "discharge Coe. "/1 -> ". "/2
  "     "/1 -> ". "/1
  ". "/1 -> " 3"/3  "mass flow actual"
  Product6/1 -> Product5/2, Sqrt1/1  "temp. correction"
  Tiso/1 -> Product6/1
  [compressor_inlet_temp] -> Product6/2
  pressure correction/1 -> "     "/1
  1 ~ 12/1 -> -1/2
  N=7250 rpm/1 -> frequency correction/2
  [rotor_freq_corr] -> frequency correction/1
  frequency correction/1 -> " 3"/2
  " 3"/1 -> Sum10/1
  [Cp_compressor_inlet] -> " 4"/2
  Sum10/1 -> time constant flow = 0.25/1
  time constant flow = 0.25/1 -> Integrator1/1
  " 4"/1 -> " 8"/2
  " 8"/1 -> Sum13/1
  Sqrt1/1 -> -1/1
  Sum7/1 -> Product5/1
  z3/1 -> Sum7/1
  IGV %/1 -> Delay = 1.2 sec/1
  Delay = 1.2 sec/1 -> Sum7/2
  MW_load/1 -> MW to kW/1
  Cp_com_in/2(Rwet) -> [R_wet]
  Mux2/1 -> k=Cp(T) /(Cp(T)-R)/1
  [Cp_compressor_inlet] -> Mux2/1
  [R_wet] -> Mux2/2
  Sum8/1 -> time constant1/1
  time constant1/1 -> Integrator2/1
  Sum13/1 -> Sum8/1
  ./1 -> Sum2/1
  Tiso1/1 -> temp. cor/2
  temp. cor/1 -> Sqrt4/1
  "pr "/1 -> 0.1 ~ 1/1
  Sum12/1 -> efficiency/1
  efficiency/1 -> Integrator3/1
  Sqrt4/1 -> "pr "/1
  Torque ----> CPR/1 -> Scope2/1, 1 ~ 12/1
  MW to kW/1 -> Product3/1
  rpm to rad/s/1 -> Product3/2
  Integrator3/1 -> [comp_perform], Scope7/1, "pr "/2, Sum12/2
  Integrator2/1 -> MW/1, [comp_conpower], Sum8/2
  Product1/1 -> " 6"/2, Cp @Cop Outlet/1(Tinlet), Sum9/1, Scope9/1, Sum3/1
  Cp @Cop Outlet/1(Cp(T)) -> " 6"/3
  " 6"/1 -> Sum13/2
  "    "/1 -> Sum9/2
  Tiso2/1 -> Product4/1
  [compressor_inlet_temp] -> Product4/2
  speed corrected/1 -> [rotor_freq_corr]
  Product4/1 -> Sqrt5/1
  Sqrt5/1 -> speed corrected/2
  [flow_cmp_out] -> " 6"/1
  Mux/1 -> Scope4/1
  Sum11/1 -> Sum14/1, Scope5/1, [flow_cmp_out], air_mass_flow/1
  0 ~ 8.5 %1/1 -> Sum5/1, Mux6/1, stator_cooling_air_flow/1
  Integrator1/1 -> Mux1/2, " 8"/1, Sum10/2, Sum11/2, " 1.5 ~ 3.2 % 1"/1, 0 ~ 8.5 %1/1
  Mux1/1 -> Scope1/1
  s/1 -> Mux1/1
  Product3/1 -> Delay = 0.85 sec/1
  Delay = 0.85 sec/1 -> Torque ----> CPR/1
  power1/1 -> MW1/1
  Mux3/1 -> Scope3/1
  s2/1 -> Mux3/1
  MW/1 -> Mux/2, comp_power/1
  Mux4/1 -> Scope6/1
  s1/1 -> Mux4/1
  -1/1 -> -/1, Mux4/2, [cmp_CPR], CPR/1
  Sum9/1 -> Mux3/2, comp_outlet_temp/1
  "    1"/1 -> Sum3/2
  Sum3/1 -> Scope8/1
  MW1/1 -> Mux/1
  Sum5/1 -> Sum14/2, Sum11/1, Mux5/2
  Mux5/1 -> Scope11/1
  s3/1 -> Mux5/1
  Mux6/1 -> Scope10/1
  " 1.5 ~ 3.2 % 1"/1 -> Sum5/2, Mux6/2, rotor_cooling_air_flow/1
  Sum14/1 -> Mux7/2
  Mux7/1 -> Scope12/1
  s4/1 -> Mux7/1
  performance correction/1 -> Memory/1
  .1/1 -> performance correction/2
  [comp_perform] -> performance correction/1
  Memory/1 -> " 3"/1

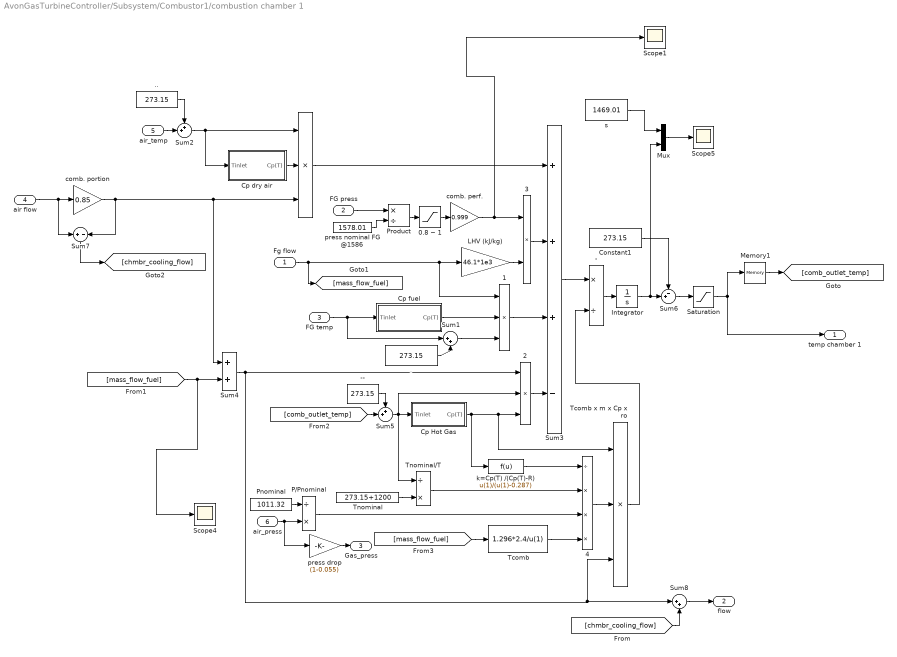
== system AvonGasTurbineController/Subsystem/Combustor1/combustion chamber 1 ==
  Fg flow : Inport
  FG press : Inport  Port=2
  FG temp : Inport  Port=3
  air flow : Inport  Port=4
  air_temp : Inport  Port=5
  air_press : Inport  Port=6
  "     " : Product  Inputs=3  RndMeth=Zero
  "     1" : Product  Inputs=3  RndMeth=Zero
  "     2" : Product  Inputs=3  RndMeth=Zero
  "     3" : Product  RndMeth=Zero
  "     4" : Product  Inputs=/***  RndMeth=Zero
  " Cp dry air " : Subsystem
  - : Product  Inputs=*/  RndMeth=Zero
  -- : Constant  Value=273.15
  . : Constant  Value=273.15
  .. : Constant  Value=273.15
  0.8 ~ 1 : Saturate  UpperLimit=1  LowerLimit=0.8
  Constant1 : Constant  Value=273.15
  "Cp Hot Gas " : Subsystem
  Cp fuel : Subsystem
  Integrator : Integrator  InitialCondition=780+273.15  LimitOutput=on  UpperSaturationLimit=2000  LowerSaturationLimit=780+273.15
  "LHV (kJ/kg) " : Gain  Gain=46.1*1e3
  Memory1 : Memory  InitialCondition=780
  Mux : Mux  Inputs=2
  P/Pnominal : Product  Inputs=/*  RndMeth=Zero
  Pnominal : Constant  Value=1011.32
  Product : Product  Inputs=*/
  Saturation : Saturate  UpperLimit=1400  LowerLimit=350
  Scope1 : Scope
  Scope4 : Scope
  Scope5 : Scope
  Sum1 : Sum  Inputs=|++
  Sum2 : Sum  Inputs=++|
  Sum3 : Sum  Inputs=+++-
  Sum4 : Sum  Inputs=2
  Sum5 : Sum  Inputs=++|
  Sum6 : Sum  Inputs=-+|
  Sum7 : Sum  Inputs=+-
  Sum8 : Sum  Inputs=|++
  Tcomb : Fcn  Expr=1.296*2.4/u(1)  SampleTime=1
  Tcomb x m x Cp x ro : Product  Inputs=3  RndMeth=Zero
  Tnominal : Constant  Value=273.15+1200
  Tnominal/T : Product  Inputs=/*  RndMeth=Zero
  comb. perf. : Gain  Gain=0.999
  comb. portion : Gain  Gain=0.85
  k=Cp(T) /(Cp(T)-R) : Fcn  Expr=u(1)/(u(1)-0.287)
  press drop : Gain  Gain=(1-0.055)  SampleTime=1
  press nominal FG @1586 : Constant  Value=1578.01
  s : Constant  Value=1469.01
  temp chamber 1 : Outport
  flow : Outport  Port=2
  Gas_press : Outport  Port=3
  wires:
  " Cp dry air "/1(Cp(T)) -> "     "/2
  ../1 -> Sum2/1
  Sum2/1 -> " Cp dry air "/1(Tinlet), "     "/1
  FG press/1 -> Product/1
  FG temp/1 -> Sum1/1, Cp fuel/1(Tinlet)
  Sum3/1 -> -/1
  Fg flow/1 -> "     1"/1, "LHV (kJ/kg) "/1, [mass_flow_fuel]
  Sum1/1 -> "     1"/3
  Cp fuel/1(Cp(T)) -> "     1"/2
  "     "/1 -> Sum3/1
  Memory1/1 -> [comb_outlet_temp]
  "     1"/1 -> Sum3/3
  ./1 -> Sum1/2
  "     2"/1 -> Sum3/4
  Tnominal/1 -> Tnominal/T/2
  Sum5/1 -> "     2"/2, "Cp Hot Gas "/1(Tinlet), Tnominal/T/1
  Constant1/1 -> Sum6/1
  Integrator/1 -> Mux/2, Sum6/2
  Sum6/1 -> Saturation/1
  "LHV (kJ/kg) "/1 -> "     3"/2
  Tcomb x m x Cp x ro/1 -> -/2
  Tnominal/T/1 -> "     4"/2
  [mass_flow_fuel] -> Scope4/1, Sum4/2
  "Cp Hot Gas "/1(Cp(T)) -> k=Cp(T) /(Cp(T)-R)/1, "     2"/3, Tcomb x m x Cp x ro/1
  --/1 -> Sum5/1
  Pnominal/1 -> P/Pnominal/1
  air_press/1 -> press drop/1, P/Pnominal/2
  "     4"/1 -> Tcomb x m x Cp x ro/2
  k=Cp(T) /(Cp(T)-R)/1 -> "     4"/1
  [comb_outlet_temp] -> Sum5/2
  P/Pnominal/1 -> "     4"/3
  air_temp/1 -> Sum2/2
  -/1 -> Integrator/1
  Saturation/1 -> temp chamber 1/1, Memory1/1
  s/1 -> Mux/1
  Sum4/1 -> "     2"/1, Sum8/1, Tcomb x m x Cp x ro/3
  Mux/1 -> Scope5/1
  press drop/1 -> Gas_press/1
  press nominal FG @1586/1 -> Product/2
  Product/1 -> 0.8 ~ 1/1
  0.8 ~ 1/1 -> comb. perf./1
  comb. perf./1 -> "     3"/1, Scope1/1
  "     3"/1 -> Sum3/2
  [mass_flow_fuel] -> Tcomb/1
  Tcomb/1 -> "     4"/4
  air flow/1 -> Sum7/1, comb. portion/1
  comb. portion/1 -> Sum7/2, "     "/3, Sum4/1
  Sum8/1 -> flow/1
  [chmbr_cooling_flow] -> Sum8/2
  Sum7/1 -> [chmbr_cooling_flow]

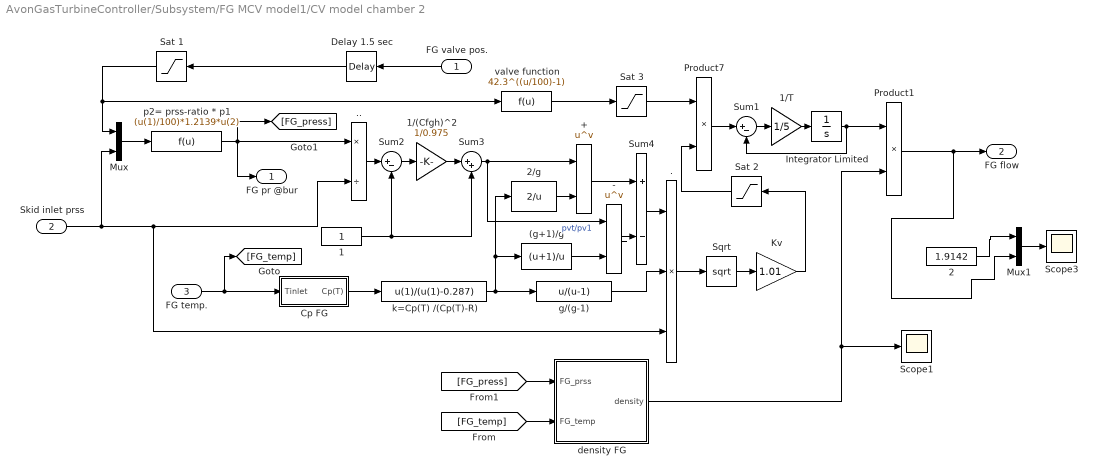
== system AvonGasTurbineController/Subsystem/FG MCV model1/CV model chamber 2 ==
  FG valve pos. : Inport
  Skid inlet prss : Inport  Port=2
  FG temp. : Inport  Port=3
  "  (g+1)/g" : Fcn  Expr=(u+1)/u
  "  Sqrt  " : Sqrt
  " k=Cp(T) /(Cp(T)-R) " : Fcn  Expr=u(1)/(u(1)-0.287)
  + : Math  Operator=pow  SignedPower=on
  - : Math  Operator=pow  SignedPower=on
  . : Product  Inputs=3  RndMeth=Zero
  .. : Product  Inputs=*/  RndMeth=Zero
  1 : Constant
  1/(Cfgh)^2 : Gain  Gain=1/0.975
  1/T : Gain  Gain=1/5
  2 : Constant  Value=1.9142
  2/g : Fcn  Expr=2/u
  Cp FG : Subsystem
  Delay 1.5 sec : TransportDelay  DelayTime=1.5  InitialOutput=30
  Integrator Limited : Integrator  InitialCondition=1.9  LimitOutput=on  UpperSaturationLimit=5  LowerSaturationLimit=0.01
  Kv : Gain  Gain=1.01
  Mux : Mux  Inputs=2
  Mux1 : Mux  Inputs=2
  Product1 : Product  RndMeth=Zero
  Product7 : Product  RndMeth=Zero
  Sat 1 : Saturate  UpperLimit=100  LowerLimit=0.01
  Sat 2 : Saturate  UpperLimit=300  LowerLimit=0.001
  Sat 3 : Saturate  UpperLimit=1  LowerLimit=0.01
  Scope1 : Scope
  Scope3 : Scope
  Sum1 : Sum  Inputs=|+-
  Sum2 : Sum  Inputs=|+-
  Sum3 : Sum  Inputs=|++
  Sum4 : Sum  Inputs=+-
  density FG : Subsystem
  g/(g-1) : Fcn  Expr=u/(u-1)
  p2= prss-ratio * p1 : Fcn  Expr=(u(1)/100)*1.2139*u(2)  SampleTime=1
  valve function : Fcn  Expr=42.3^((u/100)-1)  SampleTime=1
  FG pr @bur : Outport
  FG flow : Outport  Port=2
  wires:
  Sat 2/1 -> Product7/2
  Sum3/1 -> +/1, -/1  "pvt/pv1"
  Sum4/1 -> ./1
  "  Sqrt  "/1 -> Kv/1
  ../1 -> Sum2/1
  Skid inlet prss/1 -> ../2, ./3, Mux/2
  2/g/1 -> +/2
  1/(Cfgh)^2/1 -> Sum3/1
  Sum2/1 -> 1/(Cfgh)^2/1
  FG temp./1 -> [FG_temp], Cp FG/1(Tinlet)
  "  (g+1)/g"/1 -> -/2
  -/1 -> Sum4/2
  " k=Cp(T) /(Cp(T)-R) "/1 -> g/(g-1)/1, "  (g+1)/g"/1, 2/g/1
  g/(g-1)/1 -> ./2
  p2= prss-ratio * p1/1 -> [FG_press], ../1, FG pr @bur/1
  +/1 -> Sum4/1
  1/1 -> Sum3/2, Sum2/2
  Cp FG/1(Cp(T)) -> " k=Cp(T) /(Cp(T)-R) "/1
  Mux/1 -> p2= prss-ratio * p1/1
  valve function/1 -> Sat 3/1
  FG valve pos./1 -> Delay 1.5 sec/1
  Delay 1.5 sec/1 -> Sat 1/1
  Sat 1/1 -> Mux/1, valve function/1
  Sat 3/1 -> Product7/1
  Kv/1 -> Sat 2/1
  Sum1/1 -> 1/T/1
  1/T/1 -> Integrator Limited/1
  Integrator Limited/1 -> Product1/1, Sum1/2
  ./1 -> "  Sqrt  "/1
  Product7/1 -> Sum1/1
  [FG_temp] -> density FG/2(FG_temp)
  [FG_press] -> density FG/1(FG_prss)
  density FG/1(density) -> Scope1/1, Product1/2
  Mux1/1 -> Scope3/1
  Product1/1 -> Mux1/2, FG flow/1
  2/1 -> Mux1/1

== system AvonGasTurbineController/Subsystem/FG MCV model1/Subsystem1 ==
  gas prss : Inport
  FG temp. : Inport  Port=2
  FG flow : Inport  Port=3
  " 2 " : Constant  Value=2
  . : Product  Inputs=3  RndMeth=Zero
  2 : Constant  Value=2
  Kf : Gain  Gain=16.8993
  Math Function5 : Math  Operator=pow  SignedPower=on
  Memory : Memory
  Sqrt : Sqrt
  Sqrt1 : Sqrt
  Sqrt2 : Sqrt
  Sum1 : Sum  Inputs=-+|
  Sum5 : Sum  Inputs=|++
  Sum9 : Sum  Inputs=|+-
  Z : Subsystem
  c4 : Constant  Value=273.15
  n flow exp. : Constant  Value=0.4835
  pressure drop 5 kPa : Constant  Value=5
  pw : Math  Operator=pow  SignedPower=on
  pw1 : Math  Operator=pow  SignedPower=on
  " FG skid inlet prss" : Outport
  skid temp : Outport  Port=2
  wires:
  pressure drop 5 kPa/1 -> Sum1/1
  Sum1/1 -> pw1/1
  Sqrt1/1 -> ./3
  Memory/1 -> Z/2(P)
  Sqrt/1 -> ./2
  Sum5/1 -> Z/1(T), Sqrt/1
  c4/1 -> Sum5/2
  Z/1(Z) -> Sqrt1/1
  Sqrt2/1 -> Memory/1, " FG skid inlet prss"/1
  Math Function5/1 -> ./1
  FG flow/1 -> Math Function5/1
  n flow exp./1 -> Math Function5/2
  pw/1 -> Sum9/2
  2/1 -> pw/2
  Sum9/1 -> Sqrt2/1
  pw1/1 -> Sum9/1
  Kf/1 -> pw/1
  ./1 -> Kf/1
  FG temp./1 -> Sum5/1, skid temp/1
  " 2 "/1 -> pw1/2
  gas prss/1 -> Sum1/2

== system AvonGasTurbineController/Subsystem/Subsystem3/Cp @ trb. input ==
  Tinlet : Inport
  Cp : Fcn  Expr=(3.355+5.75*1e-4*u(1)-1600*u(1)^(-2))*0.28714  SampleTime=1
  Cp(T) : Outport
  wires:
  Cp/1 -> Cp(T)/1
  Tinlet/1 -> Cp/1

== system AvonGasTurbineController/Subsystem/Subsystem3/Cp @ trb. output ==
  Tinlet : Inport
  Cp : Fcn  Expr=(3.355+5.75*1e-4*u(1)-1600*u(1)^(-2))*0.28714  SampleTime=1
  Cp(T) : Outport
  wires:
  Tinlet/1 -> Cp/1
  Cp/1 -> Cp(T)/1

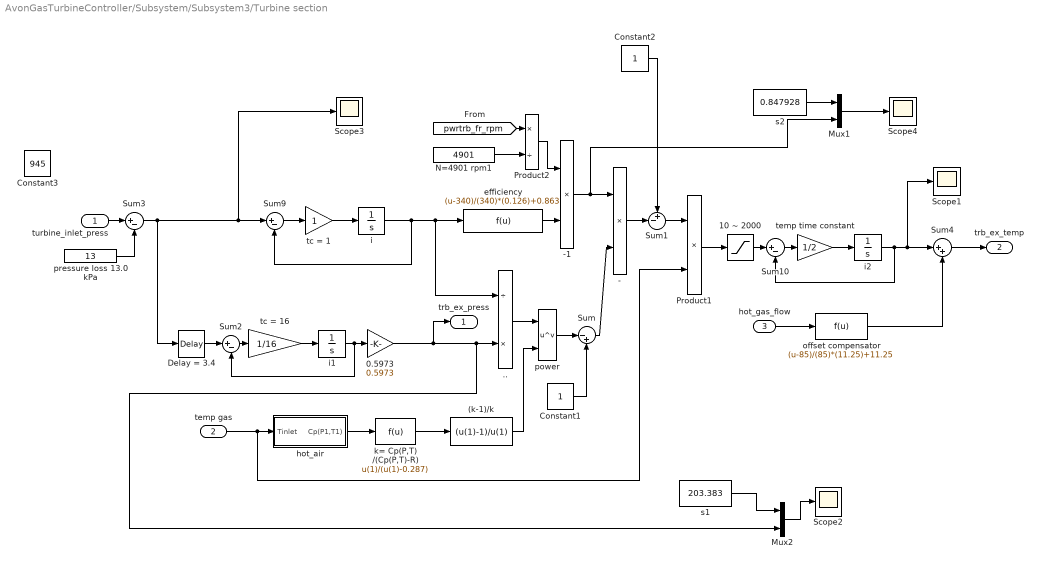
== system AvonGasTurbineController/Subsystem/Subsystem3/Turbine section ==
  turbine_inlet_press : Inport
  temp gas : Inport  Port=2
  hot_gas_flow : Inport  Port=3
  (k-1)/k : Fcn  Expr=(u(1)-1)/u(1)
  - : Product  RndMeth=Zero
  -1 : Product  RndMeth=Zero
  .. : Product  Inputs=/*  RndMeth=Zero
  0.5973 : Gain  Gain=0.5973
  10 ~ 2000 : Saturate  UpperLimit=2000  LowerLimit=10
  Constant1 : Constant
  Constant2 : Constant
  Constant3 : Constant  Value=945
  Delay = 3.4 : TransportDelay  DelayTime=3.4  InitialOutput=230.380
  Mux1 : Mux  Inputs=2
  Mux2 : Mux  Inputs=2
  N=4901 rpm1 : Constant  Value=4901
  Product1 : Product  RndMeth=Zero
  Product2 : Product  Inputs=*/  RndMeth=Zero
  Scope{1..4} (4 alike) : Scope
  Sum : Sum  Inputs=|-+
  Sum1 : Sum  Inputs=+-|
  Sum{2..3,9..10} (4 alike) : Sum  Inputs=|+-
  Sum4 : Sum  Inputs=|++
  efficiency : Fcn  Expr=(u-340)/(340)*(0.126)+0.863
  hot_air : Subsystem
  i : Integrator  InitialCondition=340  LimitOutput=on  UpperSaturationLimit=1000  LowerSaturationLimit=1
  i1 : Integrator  InitialCondition=203  LimitOutput=on  UpperSaturationLimit=500  LowerSaturationLimit=1
  i2 : Integrator  InitialCondition=1082  LimitOutput=on  UpperSaturationLimit=2000  LowerSaturationLimit=400
  k= Cp(P,T) /(Cp(P,T)-R) : Fcn  Expr=u(1)/(u(1)-0.287)
  offset compensator : Fcn  Expr=(u-85)/(85)*(11.25)+11.25  SampleTime=1
  power : Math  Operator=pow  SignedPower=on
  pressure loss 13.0 kPa : Constant  Value=13
  s1 : Constant  Value=203.383
  s2 : Constant  Value=0.847928
  tc = 1 : Gain
  tc = 16 : Gain  Gain=1/16
  temp time constant : Gain  Gain=1/2
  trb_ex_press : Outport
  trb_ex_temp : Outport  Port=2
  wires:
  ../1 -> power/1
  turbine_inlet_press/1 -> Sum3/1
  tc = 16/1 -> i1/1
  Sum2/1 -> tc = 16/1
  i1/1 -> 0.5973/1, Sum2/2
  s2/1 -> Mux1/1
  Mux1/1 -> Scope4/1
  i2/1 -> Sum10/2, Sum4/1, Scope1/1
  10 ~ 2000/1 -> Sum10/1
  temp gas/1 -> hot_air/1(Tinlet), Product1/2
  Sum1/1 -> Product1/1
  Constant2/1 -> Sum1/1
  pressure loss 13.0 kPa/1 -> Sum3/2
  Product1/1 -> 10 ~ 2000/1
  temp time constant/1 -> i2/1
  Sum10/1 -> temp time constant/1
  tc = 1/1 -> i/1
  Sum9/1 -> tc = 1/1
  Sum/1 -> -/2
  (k-1)/k/1 -> power/2
  hot_air/1(Cp(P1,T1)) -> k= Cp(P,T) /(Cp(P,T)-R)/1
  k= Cp(P,T) /(Cp(P,T)-R)/1 -> (k-1)/k/1
  Sum3/1 -> Sum9/1, Scope3/1, Delay = 3.4/1
  -/1 -> Sum1/2
  Constant1/1 -> Sum/2
  power/1 -> Sum/1
  i/1 -> efficiency/1, ../1, Sum9/2
  s1/1 -> Mux2/1
  Mux2/1 -> Scope2/1
  offset compensator/1 -> Sum4/2
  hot_gas_flow/1 -> offset compensator/1
  Sum4/1 -> trb_ex_temp/1
  0.5973/1 -> trb_ex_press/1, Mux2/2, ../2
  N=4901 rpm1/1 -> Product2/2
  [pwrtrb_fr_rpm] -> Product2/1
  Product2/1 -> -1/1
  efficiency/1 -> -1/2
  -1/1 -> Mux1/2, -/1
  Delay = 3.4/1 -> Sum2/1

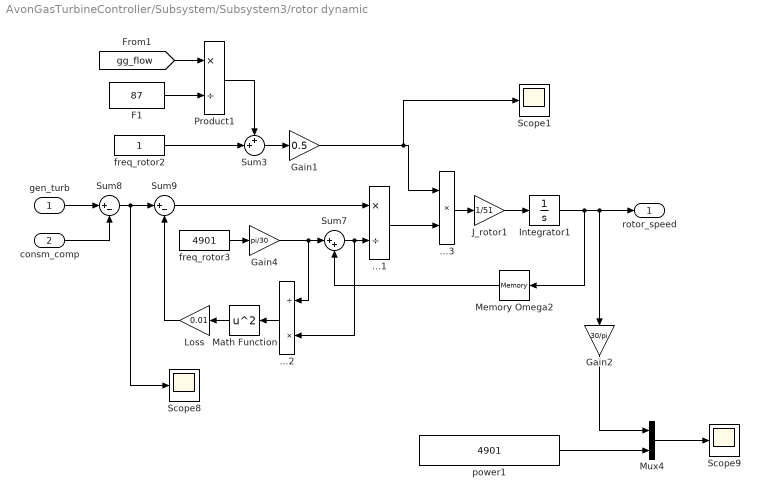
== system AvonGasTurbineController/Subsystem/Subsystem3/rotor dynamic ==
  gen_turb : Inport
  consm_comp : Inport  Port=2
  ...1 : Product  Inputs=*/
  ...2 : Product  Inputs=/*
  ...3 : Product
  F1 : Constant  Value=87
  Gain1 : Gain  Gain=0.5
  Gain2 : Gain  Gain=30/pi
  Gain4 : Gain  Gain=pi/30
  Integrator1 : Integrator  InitialCondition=pi/30*4901  LimitOutput=on  UpperSaturationLimit=4900*1.20  LowerSaturationLimit=0.01
  J_rotor1 : Gain  Gain=1/51
  Loss : Gain  Gain=0.01
  Math Function : Math  Operator=square  SignedPower=on
  Memory Omega2 : Memory  InitialCondition=pi/30*4901
  Mux4 : Mux  Inputs=2
  Product1 : Product  Inputs=*/
  Scope1 : Scope
  Scope8 : Scope
  Scope9 : Scope
  Sum3 : Sum  Inputs=++|
  Sum7 : Sum  Inputs=|++
  Sum8 : Sum  Inputs=|+-
  Sum9 : Sum  Inputs=|+-
  freq_rotor2 : Constant
  freq_rotor3 : Constant  Value=4901
  power1 : Constant  Value=4901
  rotor_speed : Outport
  wires:
  Sum9/1 -> ...1/1
  Memory Omega2/1 -> Sum7/2
  Gain4/1 -> ...2/1, Sum7/1
  Sum7/1 -> ...2/2, ...1/2
  ...3/1 -> J_rotor1/1
  ...1/1 -> ...3/2
  J_rotor1/1 -> Integrator1/1
  Loss/1 -> Sum9/2
  consm_comp/1 -> Sum8/2
  Sum8/1 -> Scope8/1, Sum9/1
  ...2/1 -> Math Function/1
  Gain1/1 -> ...3/1, Scope1/1
  Math Function/1 -> Loss/1
  Integrator1/1 -> Memory Omega2/1, rotor_speed/1, Gain2/1
  power1/1 -> Mux4/2
  Mux4/1 -> Scope9/1
  Gain2/1 -> Mux4/1
  gen_turb/1 -> Sum8/1
  freq_rotor3/1 -> Gain4/1
  F1/1 -> Product1/2
  [gg_flow] -> Product1/1
  Product1/1 -> Sum3/1
  freq_rotor2/1 -> Sum3/2
  Sum3/1 -> Gain1/1

== system AvonGasTurbineController/Subsystem/Subsystem4/Cp @ trb. input ==
  Tinlet : Inport
  Cp : Fcn  Expr=(3.355+5.75*1e-4*u(1)-1600*u(1)^(-2))*0.28714  SampleTime=1
  Cp(T) : Outport
  wires:
  Tinlet/1 -> Cp/1
  Cp/1 -> Cp(T)/1

== system AvonGasTurbineController/Subsystem/Subsystem4/Cp @ trb. output ==
  Tinlet : Inport
  Cp : Fcn  Expr=(3.355+5.75*1e-4*u(1)-1600*u(1)^(-2))*0.28714  SampleTime=1
  Cp(T) : Outport
  wires:
  Cp/1 -> Cp(T)/1
  Tinlet/1 -> Cp/1

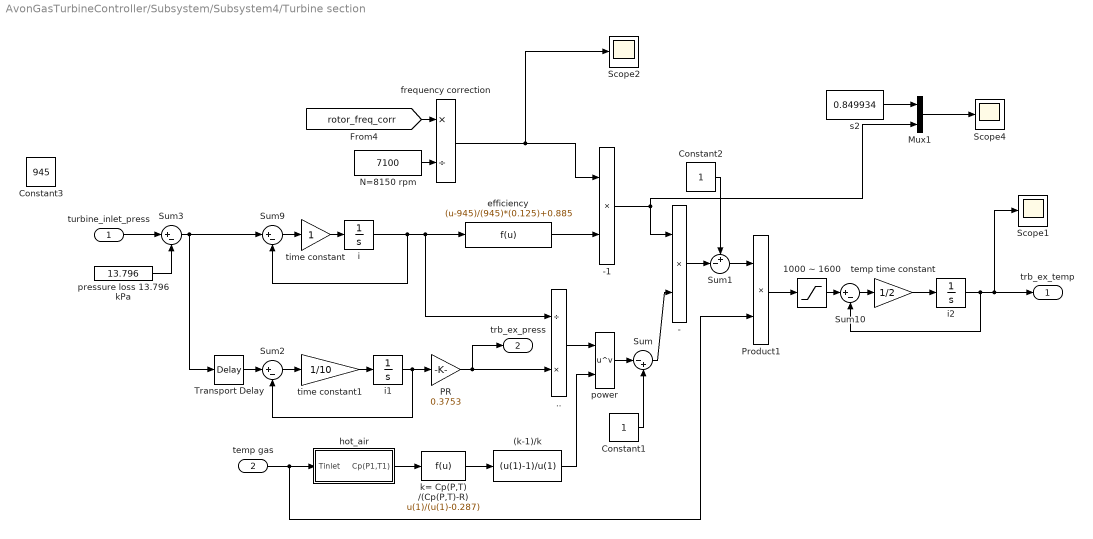
== system AvonGasTurbineController/Subsystem/Subsystem4/Turbine section ==
  turbine_inlet_press : Inport
  temp gas : Inport  Port=2
  (k-1)/k : Fcn  Expr=(u(1)-1)/u(1)
  - : Product  RndMeth=Zero
  -1 : Product  RndMeth=Zero
  .. : Product  Inputs=/*  RndMeth=Zero
  1000 ~ 1600 : Saturate  UpperLimit=2000  LowerLimit=400
  Constant1 : Constant
  Constant2 : Constant
  Constant3 : Constant  Value=945
  Mux1 : Mux  Inputs=2
  N=8150 rpm : Constant  Value=7100
  PR : Gain  Gain=0.3753
  Product1 : Product  RndMeth=Zero
  Scope1 : Scope
  Scope2 : Scope
  Scope4 : Scope
  Sum : Sum  Inputs=|-+
  Sum1 : Sum  Inputs=+-|
  Sum{2..3,9..10} (4 alike) : Sum  Inputs=|+-
  Transport Delay : TransportDelay  DelayTime=1.6  InitialOutput=941.9108
  efficiency : Fcn  Expr=(u-945)/(945)*(0.125)+0.885
  frequency correction : Product  Inputs=*/  RndMeth=Zero
  hot_air : Subsystem
  i : Integrator  InitialCondition=507  LimitOutput=on  UpperSaturationLimit=1100  LowerSaturationLimit=10
  i1 : Integrator  InitialCondition=507  LimitOutput=on  UpperSaturationLimit=1100  LowerSaturationLimit=500
  i2 : Integrator  InitialCondition=450+273.15  LimitOutput=on  UpperSaturationLimit=2000  LowerSaturationLimit=400
  k= Cp(P,T) /(Cp(P,T)-R) : Fcn  Expr=u(1)/(u(1)-0.287)
  power : Math  Operator=pow  SignedPower=on
  pressure loss 13.796 kPa : Constant  Value=13.796
  s2 : Constant  Value=0.849934
  temp time constant : Gain  Gain=1/2
  time constant : Gain
  time constant1 : Gain  Gain=1/10
  trb_ex_temp : Outport
  trb_ex_press : Outport  Port=2
  wires:
  i/1 -> Sum9/2, efficiency/1, ../1
  power/1 -> Sum/1
  Constant1/1 -> Sum/2
  -/1 -> Sum1/2
  Sum3/1 -> Sum9/1, Transport Delay/1
  k= Cp(P,T) /(Cp(P,T)-R)/1 -> (k-1)/k/1
  hot_air/1(Cp(P1,T1)) -> k= Cp(P,T) /(Cp(P,T)-R)/1
  (k-1)/k/1 -> power/2
  Sum/1 -> -/2
  Sum9/1 -> time constant/1
  time constant/1 -> i/1
  Sum10/1 -> temp time constant/1
  temp time constant/1 -> i2/1
  Product1/1 -> 1000 ~ 1600/1
  pressure loss 13.796 kPa/1 -> Sum3/2
  Constant2/1 -> Sum1/1
  Sum1/1 -> Product1/1
  temp gas/1 -> hot_air/1(Tinlet), Product1/2
  1000 ~ 1600/1 -> Sum10/1
  i2/1 -> Scope1/1, trb_ex_temp/1, Sum10/2
  Mux1/1 -> Scope4/1
  s2/1 -> Mux1/1
  -1/1 -> -/1, Mux1/2
  i1/1 -> Sum2/2, PR/1
  Sum2/1 -> time constant1/1
  time constant1/1 -> i1/1
  turbine_inlet_press/1 -> Sum3/1
  PR/1 -> trb_ex_press/1, ../2
  ../1 -> power/1
  Transport Delay/1 -> Sum2/1
  N=8150 rpm/1 -> frequency correction/2
  [rotor_freq_corr] -> frequency correction/1
  efficiency/1 -> -1/2
  frequency correction/1 -> Scope2/1, -1/1
